simulink model "TP4_reprise_commande_des_clignotants_StateFlow"  (R2022b)
settings: Solver=VariableStepAuto  StartTime=0.0  StopTime=inf  RelTol=1e-3
libraries: dspswit3 x1, simulink x1
settings Model: Creator=HP  LastModifiedBy=HP

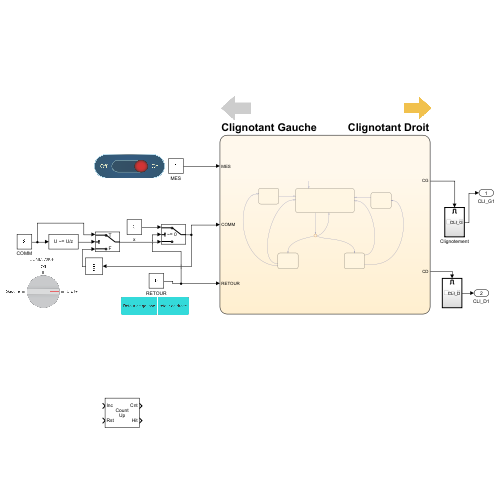
[thumbnail: Simulink's stored preview of the top-level diagram]
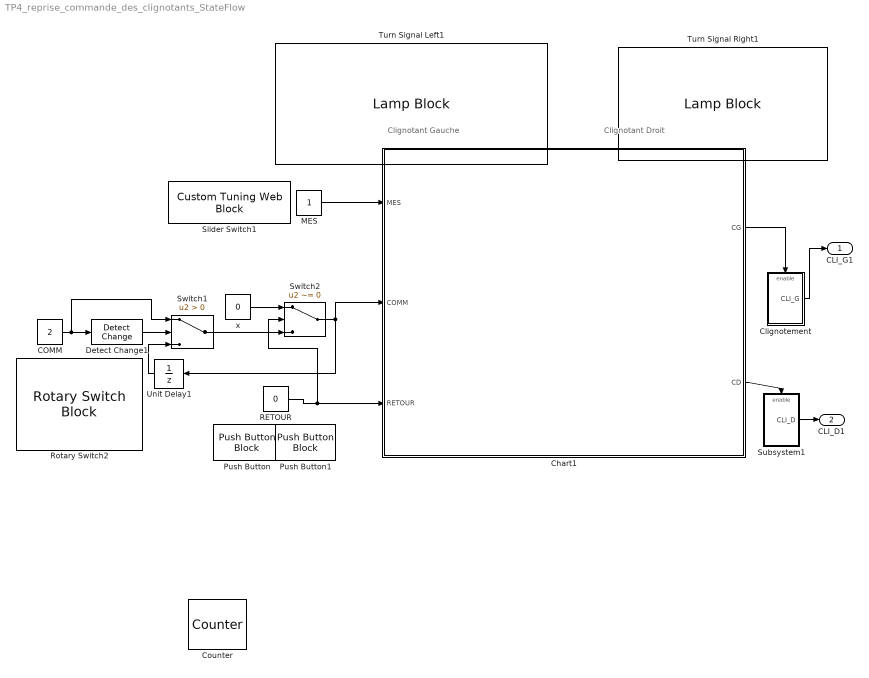
== system TP4_reprise_commande_des_clignotants_StateFlow ==
  note: Clignotant Gauche
  note: Clignotant Droit
  COMM : Constant  Value=2
  Chart1 : Stateflow chart  TreatAsAtomicUnit=on
  Clignotement : Subsystem
  Counter : dspswit3/Counter  Direction=Up  CountEvent=Rising edge  CounterSize=User defined  MaxCount=255  InitialCount=0  Output=Count and Hit  HitValue=32  ResetInput=on  SamplesPerFrame=1  Ts=1  CntDtype=double  HitDtype=Logical
  Detect Change1 : simulink/Logic and Bit Operations/Detect Change  vinit=0  OutDataTypeStr=boolean
  MES : Constant
  Push Button : PushButtonBlock  ButtonText=Retour de gauche  OnValue=2  OffValue=0.000000
  Push Button1 : PushButtonBlock  ButtonText=retour de droite  OffValue=0.000000
  RETOUR : Constant  Value=0
  Rotary Switch2 : RotarySwitchBlock
      settings: Values={{'Gauche', 'Off', 'Droite'}, [1 0 2]}
  Slider Switch1 : CustomTuningWebBlock  LabelPosition=Hide  ShowInitialText=on  Configuration="{\"type\":\"Switch\",\"settings\":{\"BindingType\":\"param\",\"backgroundColor\":[0,0,255,\"1\"],\"backgroundOffset\":0.14,\"fixedAspectRatio\":\"on\",\"foregroundColor\":[234,234,234],\"showBackgroundColor\":false,\"variant\":\"slider\"},\"components\":[{\"name\":\"CustomSwitchStateComponent\",\"settings\":{\"position\":[0,0,1,1],\"states\":[{\"HitRegion\":{\"position\":[0,0,0.5,1]},\"Image\":{\"position\":[0,0,1,1],\"size\":[1,1],\"src\":\"data:image/svg+xml;base64,PD94bWwgdmVyc2lvbj0iMS4wIiBlbmNvZGluZz0idXRmLTgiPz4NCjwhLS0gR2VuZXJhdG9yOiBBZG9iZSBJbGx1c3RyYXRvciAyNS4yLjEsIFNWRyBFeHBvcnQgUGx1Zy1JbiAuIFNWRyBWZXJzaW9uOiA2LjAwIEJ1aWxkIDApICAtLT4NCjxzdmcgdmVyc2lvbj0iMS4xIiB4bWxucz0iaHR0cDovL3d3dy53My5vcmcvMjAwMC9zdmciIHhtbG5zOnhsaW5rPSJodHRwOi8vd3d3LnczLm9yZy8xOTk5L3hsaW5rIiB4PSIwcHgiIHk9IjBweCINCgkgdmlld0JveD0iMCAwIDc2IDI5IiBzdHlsZT0iZW5hYmxlLWJhY2tncm91bmQ6bmV3 ...(+5404 chars)\",\"srcOrientation\":\"Right\"},\"Label\":{\"color\":[0.9882352941176471,0.9882352941176471,0.7725490196078432],\"icon\":{\"size\":[0,0],\"src\":[],\"srcOrientation\":\"Right\"},\"iconPlacement\":\"left\",\"opacity\":1,\"position\":[0.5,0.14],\"show\":true,\"text\":{\"content\":\"Off\",\"font\":\"Helvetica\",\"fontSize\":17.5}},\"Value\":0},{\"HitRegion\":{\"position\":[0,0.5,0.5,1]},\"Image\":{\"position\":[0,0,1,1],\"size\":[1,1],\"src\":\"data:image/svg+xml;base64,PD94bWwgdmVyc2lvbj0iMS4wIiBlbmNvZGluZz0idXRmLTgiPz4NCjwhLS0gR2VuZXJhdG9yOiBBZG9iZSBJbGx1c3RyYXRvciAyNS4yLjEsIFNWRyBFeHBvcnQgUGx1Zy1JbiAuIFNWRyBWZXJzaW9uOiA2LjAwIEJ1aWxkIDApICAtLT4NCjxzdmcgdmVyc2lvbj0iMS4xIiB4bWxucz0iaHR0cDovL3d3dy53My5vcmcvMjAwMC9zdmciIHhtbG5zOnhsaW5rPSJodHRwOi8vd3d3LnczLm9yZy8xOTk5L3hsaW5rIiB4PSIwcHgiIHk9IjBweCINCgkgdmlld0JveD0iMCAwIDc2IDI5IiBzdHlsZT0iZW5hYmxlLWJhY2tncm91bmQ6bmV3 ...(+5404 chars)\",\"srcOrientation\":\"Right\"},\"Label\":{\"color\":[0.9882352941176471,0.9882352941176471,0.7725490196078432],\"icon\":{\"size\":[0,0],\"src\":[],\"srcOrientation\":\"Right\"},\"iconPlacement\":\"left\",\"opacity\":1,\"position\":[0.5,0.86],\"show\":true,\"text\":{\"content\":\"On\",\"font\":\"Helvetica\",\"fontSize\":17.5}},\"Value\":1}]}},{\"name\":\"BackgroundImageComponent\",\"settings\":{\"image\":{\"size\":[140,55],\"src\":\"default\",\"srcOrientation\":\"Right\"},\"position\":[0,0,1,1],\"scaleMode\":\"0\"}},{\"name\":\"ForegroundImageComponent\",\"settings\":{\"image\":{\"size\":[0,0],\"src\":\"default\",\"srcOrientation\":[]},\"isForeground\":1,\"position\":[0,0,1,1],\"scaleMode\":\"0\"}}]}"
  Subsystem1 : Subsystem
  Switch1 : Switch  Criteria=u2 > Threshold  SaturateOnIntegerOverflow=off  InputSameDT=off
  Switch2 : Switch  Criteria=u2 ~= 0  SaturateOnIntegerOverflow=off  InputSameDT=off
  Turn Signal Left1 : LampBlock  LabelPosition=Hide  Icon=TurnSignalLeft
  Turn Signal Right1 : LampBlock  LabelPosition=Hide  Icon=TurnSignalRight
  Unit Delay1 : UnitDelay  SampleTime=-1  HasFrameUpgradeWarning=on
  x : Constant  Value=0
  CLI_G1 : Outport
  CLI_D1 : Outport  Port=2
  wires:
  Clignotement/1(CLI_G) -> CLI_G1/1
  Subsystem1/1(CLI_D) -> CLI_D1/1
  Switch1/1 -> Switch2/3
  x/1 -> Switch2/1
  Switch2/1 -> Unit Delay1/1, Chart1/2(COMM)
  MES/1 -> Chart1/1(MES)
  RETOUR/1 -> Chart1/3(RETOUR), Switch2/2
  Chart1/1(CG) -> Clignotement/Enable
  Chart1/2(CD) -> Subsystem1/Enable
  Detect Change1/1 -> Switch1/2
  COMM/1 -> Switch1/1, Detect Change1/1
  Unit Delay1/1 -> Switch1/3

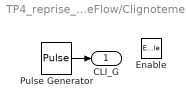
== system TP4_reprise_commande_des_clignotants_StateFlow/Clignotement ==
  Enable : EnablePort
  Pulse Generator : DiscretePulseGenerator  PulseType=Time based  Period=1  PulseWidth=50  SampleTime=-1  VectorParams1D=off
  CLI_G : Outport
  wires:
  Pulse Generator/1 -> CLI_G/1

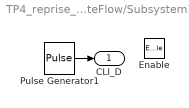
== system TP4_reprise_commande_des_clignotants_StateFlow/Subsystem1 ==
  Enable : EnablePort
  Pulse Generator1 : DiscretePulseGenerator  PulseType=Time based  Period=1  PulseWidth=50
  CLI_D : Outport
  wires:
  Pulse Generator1/1 -> CLI_D/1

== stateflow chart TP4_reprise_commande_des_clignotants_StateFlow/Chart1 ==
  state Repos2
    during:
    CG = 0;
    CD = 0;
  state initial
    entry:
    CG = 0;
    CD = 0;
  state Repos1
    entry:
    CG = 0;
    CD = 0;
  state CLI_G_activ
    entry:
    CG = 1;
    CD = 0;
  state CLI_D_activ
    entry:
    CG = 0;
    CD = 1;
  (default) -> initial
  CLI_G_activ -> Repos2 [order 2] : [after(10, sec)]
  Repos2 -> initial : [COMM == 0]
  Repos1 -> initial : [COMM == 0]
  CLI_G_activ -> initial [order 1] : [RETOUR == 1 || COMM ~= 1 || MES ~= 1]
  CLI_D_activ -> Repos1 [order 2] : [after(10, sec)]
  CLI_D_activ -> initial [order 1] : [COMM ~=2 || MES ~= 1 || RETOUR == 2]
  initial -> (junction 10) : [MES == 1]
  (junction 10) -> initial [order 2] : [MES == 0]
  (junction 10) -> CLI_G_activ [order 1] : [COMM == 1 && RETOUR ~= 1]
  (junction 10) -> CLI_D_activ [order 3] : [COMM == 2 && RETOUR ~= 2]
  data: MES input; COMM input; RETOUR input; CG output; CD output
